simulink model "ASM_Traffic_MultiCore"  (R2026a)
settings: Solver=ode1  StartTime=SIM.tstart.v  StopTime=SIM.tend.v  FixedStep=SIM.StepSize.v
PostLoadFcn:
  | if any(exist('dsrtsu_mdlpostloadfcn', 'file') ~= 0), dsrtsu_mdlpostloadfcn('Execute', bdroot); end
  | try, asm_mdl_postloadfcn(bdroot, 'UpdateModel', 3600); catch, disp(lasterr); end,
InitFcn:
  | , if any(exist('rtifpga_mdlclblib', 'file') ~= 0), rtifpga_mdlclblib('Init', bdroot); end,
  | , if any(exist('dsmpb_private', 'file') ~= 0), dsmpb_private('dsmpb_mdlclblib', 'Init', bdroot); end,
model workspace (MAT data in the model file):
  asmReferencePath = [0 0.01 0.02 0.03 0.04 0.05 0.06 0.07 0.08 0.09 0.1 0.11 ... (350007 elements, 50001x7)]
  roadBounds : Simulink.Parameter (value not decoded)
  safetyAxes : Simulink.Parameter (value not decoded)
undefined symbols (not defined in the file): _to_, a0b2, ASM_BrakeHydraulics_DemoSystems, ASM_VehicleDynamics_DemoSystems, b98103fe8ad365046cd0, BrakeCircuit, controllerConfig, CPT, Crankshaft, DiscIntNeverNeededParam, dsmsi, FinalDriveAssembly, MDL, ModeSignals, mu, Pos_BrakePedal_Maneuver, rad, RefSignals, roadFamilyData, roadFamilyId, s_to_rpm, SIM, SoftECU, Suspension, Tire, Transmission
libraries: ASM_Traffic_lib x135, simulink x98, ASM_Utils_lib x77, ASM_VehicleDynamics_lib x70, ASM_Environment_lib x22, dsmpblib x20, dsmsilib x15, MDLD_Utils_lib x10, ASM_BrakeHydraulics_lib x3, sl_discontinuities x2
(part 58 of 65)

== system ASM_Traffic_MultiCore/Environment/Sensors/PlantModel/Object_Sensor_2D/ObjectData/Sensor6/Object_Custom_Values ==
  TrafficObject_Type[] : Inport
  TrafficObject_Type_Data[] : Inport  Port=2
  CUSTOM_SENSOR_OUTPUT : ASM_Traffic_lib/Sensors/Custom_Sensor/CUSTOM_SENSOR_OUTPUT  Tag=ASM_SUBCOMPONENT  ASMProperties=struct('Name','CUSTOM_SENSOR_OUTPUT','Version','5.0','Library','ASM_Traffic_lib')  ASMInstanceName=custom_sensor_output  ASMInstanceID=26
      settings: AttributesFormatString=Instance Name: %<ASMInstanceName>\nInstance ID: %<ASMInstanceID>
  CUSTOM_SENSOR_OUTPUT1 : ASM_Traffic_lib/Sensors/Custom_Sensor/CUSTOM_SENSOR_OUTPUT  Tag=ASM_SUBCOMPONENT  ASMProperties=struct('Name','CUSTOM_SENSOR_OUTPUT','Version','5.0','Library','ASM_Traffic_lib')  ASMInstanceName=custom_sensor_output  ASMInstanceID=27
      settings: AttributesFormatString=Instance Name: %<ASMInstanceName>\nInstance ID: %<ASMInstanceID>
  CUSTOM_SENSOR_OUTPUT2 : ASM_Traffic_lib/Sensors/Custom_Sensor/CUSTOM_SENSOR_OUTPUT  Tag=ASM_SUBCOMPONENT  ASMProperties=struct('Name','CUSTOM_SENSOR_OUTPUT','Version','5.0','Library','ASM_Traffic_lib')  ASMInstanceName=custom_sensor_output  ASMInstanceID=28
      settings: AttributesFormatString=Instance Name: %<ASMInstanceName>\nInstance ID: %<ASMInstanceID>
  Terminator : Terminator
  Terminator1 : Terminator
  Terminator2 : Terminator
  Vectorize_Signals : Subsystem
  "[11:15]" : Selector  IndexOptions=Index vector (dialog)  Indices=[11:15]  OutputSizes=1
  "[1:5]" : Selector  IndexOptions=Index vector (dialog)  Indices=[1:5]  OutputSizes=1
  "[6:10]" : Selector  IndexOptions=Index vector (dialog)  Indices=[6:10]  OutputSizes=1
  Object_Custom_Values[] : Outport  VectorParamsAs1DForOutWhenUnconnected=off
  wires:
  CUSTOM_SENSOR_OUTPUT2/2 -> Vectorize_Signals/3(SensorOutput3)
  CUSTOM_SENSOR_OUTPUT1/2 -> Vectorize_Signals/2(SensorOutput2)
  Vectorize_Signals/1(Vectorized_Custom_Values) -> Object_Custom_Values[]/1
  CUSTOM_SENSOR_OUTPUT/2 -> Vectorize_Signals/1(SensorOutput1)
  CUSTOM_SENSOR_OUTPUT2/1 -> Terminator2/1
  CUSTOM_SENSOR_OUTPUT1/1 -> Terminator1/1
  CUSTOM_SENSOR_OUTPUT/1 -> Terminator/1
  "[6:10]"/1 -> CUSTOM_SENSOR_OUTPUT1/1
  TrafficObject_Type[]/1 -> "[11:15]"/1, "[6:10]"/1, "[1:5]"/1
  TrafficObject_Type_Data[]/1 -> CUSTOM_SENSOR_OUTPUT2/2, CUSTOM_SENSOR_OUTPUT1/2, CUSTOM_SENSOR_OUTPUT/2
  "[1:5]"/1 -> CUSTOM_SENSOR_OUTPUT/1
  "[11:15]"/1 -> CUSTOM_SENSOR_OUTPUT2/1

== system ASM_Traffic_MultiCore/Environment/Sensors/PlantModel/Object_Sensor_2D/ObjectData/Sensor7/ASMSignalCollector ==
  Object_Positions : Inport
  Object_Properties_Box : Inport  Port=2
  Object_Custom_Values : Inport  Port=3
  Bus Creator1 : BusCreator  Inputs=3
  Bus Selector : BusSelector  OutputSignals=Object_Positions
  Bus Selector1 : BusSelector  OutputSignals=Object_Properties_Box
  ASMSignalBus : Outport  VectorParamsAs1DForOutWhenUnconnected=off
  wires:
  Object_Positions/1 -> Bus Selector/1
  Object_Custom_Values/1 -> Bus Creator1/3
  Bus Creator1/1 -> ASMSignalBus/1  "ObjectData"
  Object_Properties_Box/1 -> Bus Selector1/1
  Bus Selector/1 -> Bus Creator1/1  "<Object_Positions>"
  Bus Selector1/1 -> Bus Creator1/2  "<Object_Properties_Box>"

== system ASM_Traffic_MultiCore/Environment/Sensors/PlantModel/Object_Sensor_2D/ObjectData/Sensor7/GetFellowPositionVector ==
  <FellowPositions> : Inport
  Bus Selector11 : BusSelector  OutputSignals=Pos_Fellows_MainPnt_CoorSys_E[x;y;z][m].Pos_x_Fellows[m],Pos_Fellows_MainPnt_CoorSys_E[x;y;z][m].Pos_y_Fellows[m],Pos_Fellows_MainPnt_CoorSys_E[x;y;z][m].Pos_z_Fellows[m],Angle_Fellows[x;y;z][deg].Angle_Roll_Fellows[deg],Angle_Fellows[x;y;z][deg].Angle_Pitch_Fellows[deg],Angle_Fellows[x;y;z][deg].Angle_Yaw_Fellows[deg]
  Mux1 : Mux  Inputs=3
  Mux2 : Mux  Inputs=3
  Pos_Fellows_MainPnt_CoorSys_E[x;y;z][m] : Outport  VectorParamsAs1DForOutWhenUnconnected=off
  Angle_Fellows[deg] : Outport  Port=2  VectorParamsAs1DForOutWhenUnconnected=off
  wires:
  Mux2/1 -> Pos_Fellows_MainPnt_CoorSys_E[x;y;z][m]/1  "Pos_Fellows_MainPnt_CoorSys_E[x;y;z][m]"
  Mux1/1 -> Angle_Fellows[deg]/1  "Pos_Fellows_MainPnt_CoorSys_E_vec"
  Bus Selector11/4 -> Mux1/1  "<Angle_Roll_Fellows[deg]>"
  Bus Selector11/1 -> Mux2/1  "<Pos_x_Fellows[m]>"
  Bus Selector11/2 -> Mux2/2  "<Pos_y_Fellows[m]>"
  Bus Selector11/6 -> Mux1/3  "<Angle_Yaw_Fellows[deg]>"
  Bus Selector11/5 -> Mux1/2  "<Angle_Pitch_Fellows[deg]>"
  <FellowPositions>/1 -> Bus Selector11/1
  Bus Selector11/3 -> Mux2/3  "<Pos_z_Fellows[m]>"

== system ASM_Traffic_MultiCore/Environment/Sensors/PlantModel/Object_Sensor_2D/ObjectData/Sensor7/Object_Custom_Values ==
  TrafficObject_Type[] : Inport
  TrafficObject_Type_Data[] : Inport  Port=2
  CUSTOM_SENSOR_OUTPUT : ASM_Traffic_lib/Sensors/Custom_Sensor/CUSTOM_SENSOR_OUTPUT  Tag=ASM_SUBCOMPONENT  ASMProperties=struct('Name','CUSTOM_SENSOR_OUTPUT','Version','5.0','Library','ASM_Traffic_lib')  ASMInstanceName=custom_sensor_output  ASMInstanceID=29
      settings: AttributesFormatString=Instance Name: %<ASMInstanceName>\nInstance ID: %<ASMInstanceID>
  CUSTOM_SENSOR_OUTPUT1 : ASM_Traffic_lib/Sensors/Custom_Sensor/CUSTOM_SENSOR_OUTPUT  Tag=ASM_SUBCOMPONENT  ASMProperties=struct('Name','CUSTOM_SENSOR_OUTPUT','Version','5.0','Library','ASM_Traffic_lib')  ASMInstanceName=custom_sensor_output  ASMInstanceID=30
      settings: AttributesFormatString=Instance Name: %<ASMInstanceName>\nInstance ID: %<ASMInstanceID>
  CUSTOM_SENSOR_OUTPUT2 : ASM_Traffic_lib/Sensors/Custom_Sensor/CUSTOM_SENSOR_OUTPUT  Tag=ASM_SUBCOMPONENT  ASMProperties=struct('Name','CUSTOM_SENSOR_OUTPUT','Version','5.0','Library','ASM_Traffic_lib')  ASMInstanceName=custom_sensor_output  ASMInstanceID=31
      settings: AttributesFormatString=Instance Name: %<ASMInstanceName>\nInstance ID: %<ASMInstanceID>
  Terminator : Terminator
  Terminator1 : Terminator
  Terminator2 : Terminator
  Vectorize_Signals : Subsystem
  "[11:15]" : Selector  IndexOptions=Index vector (dialog)  Indices=[11:15]  OutputSizes=1
  "[1:5]" : Selector  IndexOptions=Index vector (dialog)  Indices=[1:5]  OutputSizes=1
  "[6:10]" : Selector  IndexOptions=Index vector (dialog)  Indices=[6:10]  OutputSizes=1
  Object_Custom_Values[] : Outport  VectorParamsAs1DForOutWhenUnconnected=off
  wires:
  "[11:15]"/1 -> CUSTOM_SENSOR_OUTPUT2/1
  "[1:5]"/1 -> CUSTOM_SENSOR_OUTPUT/1
  TrafficObject_Type_Data[]/1 -> CUSTOM_SENSOR_OUTPUT1/2, CUSTOM_SENSOR_OUTPUT2/2, CUSTOM_SENSOR_OUTPUT/2
  TrafficObject_Type[]/1 -> "[11:15]"/1, "[6:10]"/1, "[1:5]"/1
  "[6:10]"/1 -> CUSTOM_SENSOR_OUTPUT1/1
  CUSTOM_SENSOR_OUTPUT/1 -> Terminator/1
  CUSTOM_SENSOR_OUTPUT1/1 -> Terminator1/1
  CUSTOM_SENSOR_OUTPUT2/1 -> Terminator2/1
  CUSTOM_SENSOR_OUTPUT/2 -> Vectorize_Signals/1(SensorOutput1)
  Vectorize_Signals/1(Vectorized_Custom_Values) -> Object_Custom_Values[]/1
  CUSTOM_SENSOR_OUTPUT1/2 -> Vectorize_Signals/2(SensorOutput2)
  CUSTOM_SENSOR_OUTPUT2/2 -> Vectorize_Signals/3(SensorOutput3)

== system ASM_Traffic_MultiCore/Environment/Sensors/PlantModel/Object_Sensor_3D/CustomPoints/Sensor1/CustomPoints ==
  Sensor_Idx[] : Inport
  Sensor_Data[] : Inport  Port=2
  Enable : EnablePort
  Bus Creator2 : BusCreator  Inputs=19
  CUSTOM_POINTS_1 : ASM_Traffic_lib/Sensors/Custom Points/CUSTOM_POINTS  Tag=ASM_SUBCOMPONENT  Sw_Visible_Points_Filter_Enable=MDL.Traffic.Sensors.CustomPoints_1.Sw_Visible_Points_Filter_Enable  Sw_Sort_Enable=MDL.Traffic.Sensors.CustomPoints_1.Sw_Sort_Enable  Sw_Sort_Attribute=MDL.Traffic.Sensors.CustomPoints_1.Sw_Sort_Attribute  Sw_Sort_Direction=MDL.Traffic.Sensors.CustomPoints_1.Sw_Sort_Direction  ASMProperties=struct('Name','CUSTOM_POINTS','Version','2.0','Library','ASM_Traffic_lib')  ASMInstanceName=custom_points  ASMInstanceID=1  Const_Output_Dimension_Objects=MDL.Traffic.Sensors.CustomPoints_1.Const_Output_Dimension_Objects  Const_Output_Dimension_Object_Points=MDL.Traffic.Sensors.CustomPoints_1.Const_Output_Dimension_Object_Points
  MODELDESK_GROUP : ASM_Utils_lib/ModelDeskInterface/MODELDESK_GROUP  MDLDGroup=Object Sensor 3D 1  ASMProperties=struct('Name','MODELDESK_GROUP','Version','1.0','Library','ASM_Utils_lib')
  Terminator : Terminator
  CustomPoint_Signals[] : Outport  OutputWhenDisabled=reset  InitialOutput=[0]  VectorParamsAs1DForOutWhenUnconnected=off
  wires:
  CUSTOM_POINTS_1/20 -> Bus Creator2/19  "Object_Type[]"
  CUSTOM_POINTS_1/19 -> Bus Creator2/18  "Object_ID[]"
  CUSTOM_POINTS_1/18 -> Bus Creator2/17  "Data_5[]"
  CUSTOM_POINTS_1/17 -> Bus Creator2/16  "Data_4[]"
  CUSTOM_POINTS_1/16 -> Bus Creator2/15  "Data_3[]"
  CUSTOM_POINTS_1/15 -> Bus Creator2/14  "Data_2[]"
  CUSTOM_POINTS_1/14 -> Bus Creator2/13  "Data_1[]"
  CUSTOM_POINTS_1/13 -> Bus Creator2/12  "Angle_Ver_CoorSys_S[deg]"
  CUSTOM_POINTS_1/12 -> Bus Creator2/11  "Angle_Hor_CoorSys_S[deg]"
  CUSTOM_POINTS_1/11 -> Bus Creator2/10  "Pos_CoorSys_E[x;y;z][m]"
  CUSTOM_POINTS_1/10 -> Bus Creator2/9  "Pos_CoorSys_S[x;y;z][m]"
  CUSTOM_POINTS_1/9 -> Bus Creator2/8  "a_CoorSys_S[x;y;z][m|s2]"
  CUSTOM_POINTS_1/8 -> Bus Creator2/7  "a_CoorSys_S[m|s2]"
  CUSTOM_POINTS_1/7 -> Bus Creator2/6  "v_CoorSys_S[x;y;z][m|s]"
  CUSTOM_POINTS_1/6 -> Bus Creator2/5  "v_CoorSys_S[m|s]"
  CUSTOM_POINTS_1/5 -> Bus Creator2/4  "Dist_CoorSys_S[m]"
  CUSTOM_POINTS_1/4 -> Bus Creator2/3  "ID[]"
  CUSTOM_POINTS_1/3 -> Bus Creator2/2  "Flag_Is_Occluded[0|1]"
  CUSTOM_POINTS_1/2 -> Bus Creator2/1  "Flag_In_Scope[0|1]"
  Bus Creator2/1 -> CustomPoint_Signals[]/1
  CUSTOM_POINTS_1/1 -> Terminator/1
  Sensor_Idx[]/1 -> CUSTOM_POINTS_1/1
  Sensor_Data[]/1 -> CUSTOM_POINTS_1/2

== system ASM_Traffic_MultiCore/Environment/Sensors/PlantModel/Object_Sensor_3D/CustomPoints/Sensor1/CustomPointsOutput ==
  SensorSchedulingEnable[0|1] : Inport
  SensorActive[0|1] : Inport  Port=2
  SensorEnable[0|1] : Inport  Port=3
  DelayPulse[0|1] : Inport  Port=4
  CustomPoints_Signals_In[] : Inport  Port=5
  CUSTOM_POINTS_SIGNALS_DELAY_1 : ASM_Traffic_lib/Sensors/Custom Points/CUSTOM_POINTS_SIGNALS_DELAY  ASMProperties=struct('Name','CUSTOM_POINTS_SIGNALS_DELAY','Version','2.0','Library','ASM_Traffic_lib')  ASMInstanceName=custom_points_signals_delay  ASMInstanceID=1
  HoldSignals : Subsystem
  Logical Operator1 : Logic  Operator=OR  AllPortsSameDT=off  OutDataTypeStr=boolean
  ResetPulse : Subsystem
  SignalBus : Subsystem
  CustomPoints_Signals_Out[] : Outport  VectorParamsAs1DForOutWhenUnconnected=off
  wires:
  ResetPulse/1(ResetPulse[0|1]) -> Logical Operator1/1, HoldSignals/1(ResetPulse[0|1]), CUSTOM_POINTS_SIGNALS_DELAY_1/1
  SensorEnable[0|1]/1 -> Logical Operator1/2
  Logical Operator1/1 -> HoldSignals/Enable
  SensorActive[0|1]/1 -> ResetPulse/2(SensorActive[0|1])
  HoldSignals/1(CustomPoints_Signals_Out[]) -> CUSTOM_POINTS_SIGNALS_DELAY_1/3
  SignalBus/1(CustomPoints_Signals_Out[]) -> CustomPoints_Signals_Out[]/1
  DelayPulse[0|1]/1 -> CUSTOM_POINTS_SIGNALS_DELAY_1/2
  CUSTOM_POINTS_SIGNALS_DELAY_1/1 -> SignalBus/1(CustomPoints_Signals_In[])
  CustomPoints_Signals_In[]/1 -> HoldSignals/2(CustomPoints_Signals_In[])
  SensorSchedulingEnable[0|1]/1 -> ResetPulse/1(Enable[0|1])

== system ASM_Traffic_MultiCore/Environment/Sensors/PlantModel/Object_Sensor_3D/CustomPoints/Sensor2/CustomPoints ==
  Sensor_Idx[] : Inport
  Sensor_Data[] : Inport  Port=2
  Enable : EnablePort
  Bus Creator2 : BusCreator  Inputs=19
  CUSTOM_POINTS_2 : ASM_Traffic_lib/Sensors/Custom Points/CUSTOM_POINTS  Tag=ASM_SUBCOMPONENT  Sw_Visible_Points_Filter_Enable=MDL.Traffic.Sensors.CustomPoints_2.Sw_Visible_Points_Filter_Enable  Sw_Sort_Enable=MDL.Traffic.Sensors.CustomPoints_2.Sw_Sort_Enable  Sw_Sort_Attribute=MDL.Traffic.Sensors.CustomPoints_2.Sw_Sort_Attribute  Sw_Sort_Direction=MDL.Traffic.Sensors.CustomPoints_2.Sw_Sort_Direction  ASMProperties=struct('Name','CUSTOM_POINTS','Version','2.0','Library','ASM_Traffic_lib')  ASMInstanceName=custom_points  ASMInstanceID=2  Const_Output_Dimension_Objects=MDL.Traffic.Sensors.CustomPoints_2.Const_Output_Dimension_Objects  Const_Output_Dimension_Object_Points=MDL.Traffic.Sensors.CustomPoints_2.Const_Output_Dimension_Object_Points
      settings: AttributesFormatString=Instance Name: %<ASMInstanceName>\nInstance ID: %<ASMInstanceID>
  MODELDESK_GROUP : ASM_Utils_lib/ModelDeskInterface/MODELDESK_GROUP  MDLDGroup=Object Sensor 3D 2  ASMProperties=struct('Name','MODELDESK_GROUP','Version','1.0','Library','ASM_Utils_lib')
  Terminator : Terminator
  CustomPoint_Signals[] : Outport  OutputWhenDisabled=reset  InitialOutput=[0]  VectorParamsAs1DForOutWhenUnconnected=off
  wires:
  CUSTOM_POINTS_2/3 -> Bus Creator2/2  "Flag_Is_Occluded[0|1]"
  CUSTOM_POINTS_2/11 -> Bus Creator2/10  "Pos_CoorSys_E[x;y;z][m]"
  CUSTOM_POINTS_2/8 -> Bus Creator2/7  "a_CoorSys_S[m|s2]"
  CUSTOM_POINTS_2/5 -> Bus Creator2/4  "Dist_CoorSys_S[m]"
  CUSTOM_POINTS_2/4 -> Bus Creator2/3  "ID[]"
  CUSTOM_POINTS_2/13 -> Bus Creator2/12  "Angle_Ver_CoorSys_S[deg]"
  CUSTOM_POINTS_2/6 -> Bus Creator2/5  "v_CoorSys_S[m|s]"
  CUSTOM_POINTS_2/7 -> Bus Creator2/6  "v_CoorSys_S[x;y;z][m|s]"
  CUSTOM_POINTS_2/15 -> Bus Creator2/14  "Data_2[]"
  CUSTOM_POINTS_2/16 -> Bus Creator2/15  "Data_3[]"
  CUSTOM_POINTS_2/14 -> Bus Creator2/13  "Data_1[]"
  CUSTOM_POINTS_2/10 -> Bus Creator2/9  "Pos_CoorSys_S[x;y;z][m]"
  CUSTOM_POINTS_2/12 -> Bus Creator2/11  "Angle_Hor_CoorSys_S[deg]"
  CUSTOM_POINTS_2/18 -> Bus Creator2/17  "Data_5[]"
  CUSTOM_POINTS_2/17 -> Bus Creator2/16  "Data_4[]"
  Bus Creator2/1 -> CustomPoint_Signals[]/1
  CUSTOM_POINTS_2/2 -> Bus Creator2/1  "Flag_In_Scope[0|1]"
  CUSTOM_POINTS_2/9 -> Bus Creator2/8  "a_CoorSys_S[x;y;z][m|s2]"
  CUSTOM_POINTS_2/19 -> Bus Creator2/18  "Object_ID[]"
  CUSTOM_POINTS_2/20 -> Bus Creator2/19  "Object_Type[]"
  Sensor_Data[]/1 -> CUSTOM_POINTS_2/2
  Sensor_Idx[]/1 -> CUSTOM_POINTS_2/1
  CUSTOM_POINTS_2/1 -> Terminator/1

== system ASM_Traffic_MultiCore/Environment/Sensors/PlantModel/Object_Sensor_3D/CustomPoints/Sensor2/CustomPointsOutput ==
  SensorSchedulingEnable[0|1] : Inport
  SensorActive[0|1] : Inport  Port=2
  SensorEnable[0|1] : Inport  Port=3
  DelayPulse[0|1] : Inport  Port=4
  CustomPoint_Signals_In[] : Inport  Port=5
  CUSTOM_POINTS_SIGNALS_DELAY_2 : ASM_Traffic_lib/Sensors/Custom Points/CUSTOM_POINTS_SIGNALS_DELAY  ASMProperties=struct('Name','CUSTOM_POINTS_SIGNALS_DELAY','Version','2.0','Library','ASM_Traffic_lib')  ASMInstanceName=custom_points_signals_delay  ASMInstanceID=1
  HoldSignals : Subsystem
  Logical Operator1 : Logic  Operator=OR  AllPortsSameDT=off  OutDataTypeStr=boolean
  ResetPulse : Subsystem
  SignalBus : Subsystem
  CustomPoints_Signals_Out[] : Outport  VectorParamsAs1DForOutWhenUnconnected=off
  wires:
  SensorActive[0|1]/1 -> ResetPulse/2(SensorActive[0|1])
  ResetPulse/1(ResetPulse[0|1]) -> Logical Operator1/1, HoldSignals/1(ResetPulse[0|1]), CUSTOM_POINTS_SIGNALS_DELAY_2/1
  SensorEnable[0|1]/1 -> Logical Operator1/2
  SensorSchedulingEnable[0|1]/1 -> ResetPulse/1(Enable[0|1])
  DelayPulse[0|1]/1 -> CUSTOM_POINTS_SIGNALS_DELAY_2/2
  Logical Operator1/1 -> HoldSignals/Enable
  HoldSignals/1(CustomPoints_Signals_Out[]) -> CUSTOM_POINTS_SIGNALS_DELAY_2/3
  SignalBus/1(CustomPoints_Signals_Out[]) -> CustomPoints_Signals_Out[]/1
  CUSTOM_POINTS_SIGNALS_DELAY_2/1 -> SignalBus/1(CustomPoints_Signals_In[])
  CustomPoint_Signals_In[]/1 -> HoldSignals/2(CustomPoints_Signals_In[])

== system ASM_Traffic_MultiCore/Environment/Sensors/PlantModel/Object_Sensor_3D/CustomPoints/Sensor3/CustomPoints ==
  Sensor_Idx[] : Inport
  Sensor_Data[] : Inport  Port=2
  Enable : EnablePort
  Bus Creator2 : BusCreator  Inputs=19
  CUSTOM_POINTS_3 : ASM_Traffic_lib/Sensors/Custom Points/CUSTOM_POINTS  Tag=ASM_SUBCOMPONENT  Sw_Visible_Points_Filter_Enable=MDL.Traffic.Sensors.CustomPoints_3.Sw_Visible_Points_Filter_Enable  Sw_Sort_Enable=MDL.Traffic.Sensors.CustomPoints_3.Sw_Sort_Enable  Sw_Sort_Attribute=MDL.Traffic.Sensors.CustomPoints_3.Sw_Sort_Attribute  Sw_Sort_Direction=MDL.Traffic.Sensors.CustomPoints_3.Sw_Sort_Direction  ASMProperties=struct('Name','CUSTOM_POINTS','Version','2.0','Library','ASM_Traffic_lib')  ASMInstanceName=custom_points  ASMInstanceID=3  Const_Output_Dimension_Objects=MDL.Traffic.Sensors.CustomPoints_3.Const_Output_Dimension_Objects  Const_Output_Dimension_Object_Points=MDL.Traffic.Sensors.CustomPoints_3.Const_Output_Dimension_Object_Points
      settings: AttributesFormatString=Instance Name: %<ASMInstanceName>\nInstance ID: %<ASMInstanceID>
  MODELDESK_GROUP : ASM_Utils_lib/ModelDeskInterface/MODELDESK_GROUP  MDLDGroup=Object Sensor 3D 3  ASMProperties=struct('Name','MODELDESK_GROUP','Version','1.0','Library','ASM_Utils_lib')
  Terminator : Terminator
  CustomPoint_Signals[] : Outport  OutputWhenDisabled=reset  InitialOutput=[0]  VectorParamsAs1DForOutWhenUnconnected=off
  wires:
  CUSTOM_POINTS_3/3 -> Bus Creator2/2  "Flag_Is_Occluded[0|1]"
  CUSTOM_POINTS_3/11 -> Bus Creator2/10  "Pos_CoorSys_E[x;y;z][m]"
  CUSTOM_POINTS_3/8 -> Bus Creator2/7  "a_CoorSys_S[m|s2]"
  CUSTOM_POINTS_3/5 -> Bus Creator2/4  "Dist_CoorSys_S[m]"
  CUSTOM_POINTS_3/4 -> Bus Creator2/3  "ID[]"
  CUSTOM_POINTS_3/13 -> Bus Creator2/12  "Angle_Ver_CoorSys_S[deg]"
  CUSTOM_POINTS_3/6 -> Bus Creator2/5  "v_CoorSys_S[m|s]"
  CUSTOM_POINTS_3/7 -> Bus Creator2/6  "v_CoorSys_S[x;y;z][m|s]"
  CUSTOM_POINTS_3/15 -> Bus Creator2/14  "Data_2[]"
  CUSTOM_POINTS_3/16 -> Bus Creator2/15  "Data_3[]"
  CUSTOM_POINTS_3/14 -> Bus Creator2/13  "Data_1[]"
  CUSTOM_POINTS_3/10 -> Bus Creator2/9  "Pos_CoorSys_S[x;y;z][m]"
  CUSTOM_POINTS_3/12 -> Bus Creator2/11  "Angle_Hor_CoorSys_S[deg]"
  CUSTOM_POINTS_3/18 -> Bus Creator2/17  "Data_5[]"
  CUSTOM_POINTS_3/17 -> Bus Creator2/16  "Data_4[]"
  Bus Creator2/1 -> CustomPoint_Signals[]/1
  CUSTOM_POINTS_3/2 -> Bus Creator2/1  "Flag_In_Scope[0|1]"
  CUSTOM_POINTS_3/9 -> Bus Creator2/8  "a_CoorSys_S[x;y;z][m|s2]"
  CUSTOM_POINTS_3/19 -> Bus Creator2/18  "Object_ID[]"
  CUSTOM_POINTS_3/20 -> Bus Creator2/19  "Object_Type[]"
  Sensor_Idx[]/1 -> CUSTOM_POINTS_3/1
  Sensor_Data[]/1 -> CUSTOM_POINTS_3/2
  CUSTOM_POINTS_3/1 -> Terminator/1

== system ASM_Traffic_MultiCore/Environment/Sensors/PlantModel/Object_Sensor_3D/CustomPoints/Sensor3/CustomPointsOutput ==
  SensorSchedulingEnable[0|1] : Inport
  SensorActive[0|1] : Inport  Port=2
  SensorEnable[0|1] : Inport  Port=3
  DelayPulse[0|1] : Inport  Port=4
  CustomPoints_Signals_In[] : Inport  Port=5
  CUSTOM_POINTS_SIGNALS_DELAY_3 : ASM_Traffic_lib/Sensors/Custom Points/CUSTOM_POINTS_SIGNALS_DELAY  ASMProperties=struct('Name','CUSTOM_POINTS_SIGNALS_DELAY','Version','2.0','Library','ASM_Traffic_lib')  ASMInstanceName=custom_points_signals_delay  ASMInstanceID=1
  HoldSignals : Subsystem
  Logical Operator1 : Logic  Operator=OR  AllPortsSameDT=off  OutDataTypeStr=boolean
  ResetPulse1 : Subsystem
  SignalBus : Subsystem
  CustomPoints_Signals_Out[] : Outport  VectorParamsAs1DForOutWhenUnconnected=off
  wires:
  DelayPulse[0|1]/1 -> CUSTOM_POINTS_SIGNALS_DELAY_3/2
  SensorActive[0|1]/1 -> ResetPulse1/2(SensorActive[0|1])
  ResetPulse1/1(ResetPulse[0|1]) -> Logical Operator1/1, HoldSignals/1(ResetPulse[0|1]), CUSTOM_POINTS_SIGNALS_DELAY_3/1
  SensorSchedulingEnable[0|1]/1 -> ResetPulse1/1(Enable[0|1])
  SensorEnable[0|1]/1 -> Logical Operator1/2
  HoldSignals/1(CustomPoints_Signals_Out[]) -> CUSTOM_POINTS_SIGNALS_DELAY_3/3
  Logical Operator1/1 -> HoldSignals/Enable
  SignalBus/1(CustomPoints_Signals_Out[]) -> CustomPoints_Signals_Out[]/1
  CUSTOM_POINTS_SIGNALS_DELAY_3/1 -> SignalBus/1(CustomPoints_Signals_In[])
  CustomPoints_Signals_In[]/1 -> HoldSignals/2(CustomPoints_Signals_In[])

== system ASM_Traffic_MultiCore/Environment/Sensors/PlantModel/Object_Sensor_3D/ObjectData/BoundingBoxData_CoorSys_E/BoundingBoxData_CoorSys_E ==
  Object_ID[] : Inport
  Object_Type[] : Inport  Port=2
  Traffic_Signals : Inport  Port=3
  Road_Signals : Inport  Port=4
  Bus Creator1 : BusCreator  Inputs=9
  Bus Selector1 : BusSelector  OutputSignals=Object_Properties_Box.Length_Object[m],Object_Properties_Box.Width_Object[m],Object_Properties_Box.Height_Object[m],Object_Properties_Box.Flag_BoxProperties[0|1]
  Bus Selector2 : BusSelector  OutputSignals=Object_Positions.Angle_x_Objects_CoorSysE[deg],Object_Positions.Angle_y_Objects_CoorSysE[deg],Object_Positions.Angle_z_Objects_CoorSysE[deg]
  Bus Selector3 : BusSelector  OutputSignals=Object_Properties_Box.PosVec_x_CenterPnt_Object[m],Object_Properties_Box.PosVec_y_CenterPnt_Object[m],Object_Properties_Box.PosVec_z_CenterPnt_Object[m]
  Bus Selector4 : BusSelector  OutputSignals=Plant.Road_TrafficFellows.Network_Item_Type_Fellows[],Plant.Road_TrafficFellows.Network_Item_Id_Fellows[],Plant.TrafficObject_Data[]
  Bus Selector5 : BusSelector  OutputSignals=Plant.Traffic_Signals_toEnvironment
  Bus Selector6 : BusSelector  OutputSignals=Plant.ObjectParameters.TrafficObjects.TrafficObject_Type_Data[]
  Bus Selector7 : BusSelector  OutputSignals=Object_Positions.Pos_x_MainPnt_Objects_CoorSysE[m],Object_Positions.Pos_y_MainPnt_Objects_CoorSysE[m],Object_Positions.Pos_z_MainPnt_Objects_CoorSysE[m]
  Bus Selector8 : BusSelector  OutputSignals=Object_Positions.Angle_x_Objects_CoorSysE[deg],Object_Positions.Angle_y_Objects_CoorSysE[deg],Object_Positions.Angle_z_Objects_CoorSysE[deg]
  COORDINATE_TRANSFORMATION_B_TO_A : ASM_Utils_lib/MatrixOperations/COORDINATE_TRANSFORMATION_B_TO_A  ASMLibrary2Check=ASM_Traffic_lib
  GetFellowPositionVector : Subsystem
  OBJECT_POSITION : ASM_Traffic_lib/Objects/OBJECT_POSITION  MaxNumFellows=MDL.Traffic.MaxNumFellows  ASMProperties=struct('Name','OBJECT_POSITION','Version','2.0','Library','ASM_Traffic_lib')  ASMInstanceName=object_position  ASMInstanceID=1
  OBJECT_PROPERTIES_BOX : ASM_Traffic_lib/Objects/OBJECT_PROPERTIES_BOX  ASMProperties=struct('Name','OBJECT_PROPERTIES_BOX','Version','2.0','Library','ASM_Traffic_lib')  ASMInstanceName=object_properties_box  ASMInstanceID=1
  Product{,1..8} (9 alike) : Product
  Terminator : Terminator
  Terminator1 : Terminator
  Boundingboxes : Outport  VectorParamsAs1DForOutWhenUnconnected=off
  wires:
  Bus Selector5/1 -> GetFellowPositionVector/1(<FellowPositions>)  "<Traffic_Signals_toEnvironment>"
  Traffic_Signals/1 -> Bus Selector6/1, Bus Selector5/1
  GetFellowPositionVector/1(Pos_Fellows_MainPnt_CoorSys_E[x;y;z][m]) -> OBJECT_POSITION/2
  GetFellowPositionVector/2(Angle_Fellows[deg]) -> OBJECT_POSITION/3
  Bus Selector1/1 -> Product6/1  "<Length_Object[m]>"
  Bus Selector1/2 -> Product7/1  "<Width_Object[m]>"
  Bus Selector1/3 -> Product8/1  "<Height_Object[m]>"
  Bus Selector1/4 -> Product7/2, Product3/2, Product2/2, Product1/2, Product/2, Product4/2, Product5/2, Product6/2, Product8/2  "<Flag_BoxProperties[0|1]>"
  Product8/1 -> Bus Creator1/9  "Height_Object[m]"
  Product7/1 -> Bus Creator1/8  "Width_Object[m]"
  Product6/1 -> Bus Creator1/7  "Length_Object[m]"
  Product5/1 -> Bus Creator1/6  "Angle_z_Objects_CoorSysE[deg]"
  Product4/1 -> Bus Creator1/5  "Angle_y_Objects_CoorSysE[deg]"
  Product3/1 -> Bus Creator1/4  "Angle_x_Objects_CoorSysE[deg]"
  Product2/1 -> Bus Creator1/3  "Pos_z_CoorSysE[m]"
  Product1/1 -> Bus Creator1/2  "Pos_y_CoorSysE[m]"
  Product/1 -> Bus Creator1/1  "Pos_x_CoorSysE[m]"
  Bus Selector8/1 -> COORDINATE_TRANSFORMATION_B_TO_A/7  "<Angle_x_Objects_CoorSysE[deg]>"
  Bus Selector8/2 -> COORDINATE_TRANSFORMATION_B_TO_A/8  "<Angle_y_Objects_CoorSysE[deg]>"
  Bus Selector8/3 -> COORDINATE_TRANSFORMATION_B_TO_A/9  "<Angle_z_Objects_CoorSysE[deg]>"
  COORDINATE_TRANSFORMATION_B_TO_A/3 -> Product2/1  "Pos_z_CoorSysE[m]"
  COORDINATE_TRANSFORMATION_B_TO_A/2 -> Product1/1  "Pos_y_CoorSysE[m]"
  COORDINATE_TRANSFORMATION_B_TO_A/1 -> Product/1  "Pos_x_CoorSysE[m]"
  Bus Selector2/3 -> Product5/1  "<Angle_z_Objects_CoorSysE[deg]>"
  Bus Selector2/2 -> Product4/1  "<Angle_y_Objects_CoorSysE[deg]>"
  Bus Selector2/1 -> Product3/1  "<Angle_x_Objects_CoorSysE[deg]>"
  Bus Selector7/3 -> COORDINATE_TRANSFORMATION_B_TO_A/3  "<Pos_z_MainPnt_Objects_CoorSysE[m]>"
  Bus Selector7/2 -> COORDINATE_TRANSFORMATION_B_TO_A/2  "<Pos_y_MainPnt_Objects_CoorSysE[m]>"
  Bus Selector7/1 -> COORDINATE_TRANSFORMATION_B_TO_A/1  "<Pos_x_MainPnt_Objects_CoorSysE[m]>"
  Bus Selector3/1 -> COORDINATE_TRANSFORMATION_B_TO_A/4  "<PosVec_x_CenterPnt_Object[m]>"
  Bus Selector3/2 -> COORDINATE_TRANSFORMATION_B_TO_A/5  "<PosVec_y_CenterPnt_Object[m]>"
  Bus Selector3/3 -> COORDINATE_TRANSFORMATION_B_TO_A/6  "<PosVec_z_CenterPnt_Object[m]>"
  Bus Creator1/1 -> Boundingboxes/1  "Boundingboxes_DetectedObjects"
  Object_Type[]/1 -> OBJECT_PROPERTIES_BOX/1
  Object_ID[]/1 -> OBJECT_POSITION/1
  OBJECT_PROPERTIES_BOX/2 -> Bus Selector1/1, Bus Selector3/1
  OBJECT_POSITION/2 -> Bus Selector8/1, Bus Selector2/1, Bus Selector7/1
  Bus Selector6/1 -> OBJECT_PROPERTIES_BOX/2  "<TrafficObject_Type_Data[]>"
  Bus Selector4/3 -> OBJECT_POSITION/6  "<TrafficObject_Data[]>"
  Bus Selector4/2 -> OBJECT_POSITION/5  "<Network_Item_Id_Fellows[]>"
  Bus Selector4/1 -> OBJECT_POSITION/4  "<Network_Item_Type_Fellows[]>"
  Road_Signals/1 -> Bus Selector4/1
  OBJECT_PROPERTIES_BOX/1 -> Terminator1/1
  OBJECT_POSITION/1 -> Terminator/1

== system ASM_Traffic_MultiCore/Environment/Sensors/PlantModel/Object_Sensor_3D/ObjectData/BoundingBoxData_CoorSys_E/Unique_Signals_Sorted ==
  Sensor1_Signals[] : Inport
  Sensor2_Signals[] : Inport  Port=2
  Sensor3_Signals[] : Inport  Port=3
  Bus Selector : BusSelector  OutputSignals=SensorOutput.Dist_Object[m]
  Bus Selector1 : BusSelector  OutputSignals=SensorOutput.Object_ID[]
  Bus Selector10 : BusSelector  OutputSignals=Info.Flag_Object_In_Scope[0Out|1In]
  Bus Selector11 : BusSelector  OutputSignals=Info.Flag_Object_In_Scope[0Out|1In]
  Bus Selector2 : BusSelector  OutputSignals=SensorOutput.Dist_Object[m]
  Bus Selector3 : BusSelector  OutputSignals=SensorOutput.Dist_Object[m]
  Bus Selector4 : BusSelector  OutputSignals=SensorOutput.Object_Type[]
  Bus Selector5 : BusSelector  OutputSignals=SensorOutput.Object_ID[]
  Bus Selector6 : BusSelector  OutputSignals=SensorOutput.Object_ID[]
  Bus Selector7 : BusSelector  OutputSignals=SensorOutput.Object_Type[]
  Bus Selector8 : BusSelector  OutputSignals=SensorOutput.Object_Type[]
  Bus Selector9 : BusSelector  OutputSignals=Info.Flag_Object_In_Scope[0Out|1In]
  DETECTED_OBJECTS_MERGE : ASM_Traffic_lib/Sensors/Utilities/DETECTED_OBJECTS_MERGE  Const_Output_Dimension=MDL.Traffic.Sensors.DetectedObjectsMerge.Const_Output_Dimension  ASMProperties=struct('Name','DETECTED_OBJECTS_MERGE','Version','1.0','Library','ASM_Traffic_lib')  ASMInstanceName=detected_objects_merge  ASMInstanceID=1
  Mux{,1..3} (4 alike) : Mux  Inputs=3
  Terminator : Terminator
  Object_ID[] : Outport  VectorParamsAs1DForOutWhenUnconnected=off
  Object_Type[] : Outport  Port=2  VectorParamsAs1DForOutWhenUnconnected=off
  wires:
  Mux3/1 -> DETECTED_OBJECTS_MERGE/1  "Flag_Object_In_Scope[0Out|1In]"
  Bus Selector10/1 -> Mux3/2  "<Flag_Object_In_Scope[0Out|1In]>"
  Bus Selector11/1 -> Mux3/3  "<Flag_Object_In_Scope[0Out|1In]>"
  Bus Selector9/1 -> Mux3/1  "<Flag_Object_In_Scope[0Out|1In]>"
  DETECTED_OBJECTS_MERGE/3 -> Object_Type[]/1
  DETECTED_OBJECTS_MERGE/2 -> Object_ID[]/1
  DETECTED_OBJECTS_MERGE/1 -> Terminator/1
  Bus Selector1/1 -> Mux1/1  "<Object_ID[]>"
  Bus Selector2/1 -> Mux/2  "<Dist_Object[m]>"
  Bus Selector3/1 -> Mux/3  "<Dist_Object[m]>"
  Bus Selector5/1 -> Mux1/2  "<Object_ID[]>"
  Bus Selector6/1 -> Mux1/3  "<Object_ID[]>"
  Bus Selector4/1 -> Mux2/1  "<Object_Type[]>"
  Bus Selector7/1 -> Mux2/2  "<Object_Type[]>"
  Bus Selector8/1 -> Mux2/3  "<Object_Type[]>"
  Sensor2_Signals[]/1 -> Bus Selector2/1, Bus Selector5/1, Bus Selector7/1, Bus Selector10/1
  Mux1/1 -> DETECTED_OBJECTS_MERGE/3  "Object_ID[]"
  Sensor1_Signals[]/1 -> Bus Selector9/1, Bus Selector/1, Bus Selector1/1, Bus Selector4/1
  Sensor3_Signals[]/1 -> Bus Selector3/1, Bus Selector8/1, Bus Selector6/1, Bus Selector11/1
  Bus Selector/1 -> Mux/1  "<Dist_Object[m]>"
  Mux2/1 -> DETECTED_OBJECTS_MERGE/4  "Object_Type[]"
  Mux/1 -> DETECTED_OBJECTS_MERGE/2  "Dist_Object[m]"

== system ASM_Traffic_MultiCore/Environment/Sensors/PlantModel/Object_Sensor_3D/ObjectData/BoundingBoxData_CoorSys_E/avoid_incomplete_trace2source ==
  In1 : Inport
  DummyGain : Gain
  Out1 : Outport
  wires:
  In1/1 -> DummyGain/1
  DummyGain/1 -> Out1/1

== system ASM_Traffic_MultiCore/Environment/Sensors/PlantModel/Object_Sensor_3D/ObjectData/BoundingBoxData_CoorSys_E/avoid_incomplete_trace2source1 ==
  In1 : Inport
  DummyGain : Gain
  Out1 : Outport
  wires:
  DummyGain/1 -> Out1/1
  In1/1 -> DummyGain/1

== system ASM_Traffic_MultiCore/Environment/Sensors/PlantModel/Object_Sensor_3D/ObjectData/Sensor1/ASMSignalCollector ==
  Object_Positions : Inport
  Object_Properties_Box : Inport  Port=2
  Object_Custom_Values : Inport  Port=3
  Bus Creator1 : BusCreator  Inputs=3
  Bus Selector : BusSelector  OutputSignals=Object_Positions
  Bus Selector1 : BusSelector  OutputSignals=Object_Properties_Box
  ASMSignalBus : Outport  VectorParamsAs1DForOutWhenUnconnected=off
  wires:
  Object_Positions/1 -> Bus Selector/1
  Object_Custom_Values/1 -> Bus Creator1/3
  Bus Creator1/1 -> ASMSignalBus/1  "ObjectData"
  Object_Properties_Box/1 -> Bus Selector1/1
  Bus Selector/1 -> Bus Creator1/1  "<Object_Positions>"
  Bus Selector1/1 -> Bus Creator1/2  "<Object_Properties_Box>"

== system ASM_Traffic_MultiCore/Environment/Sensors/PlantModel/Object_Sensor_3D/ObjectData/Sensor1/GetFellowPositionVector ==
  <FellowPositions> : Inport
  Bus Selector11 : BusSelector  OutputSignals=Pos_Fellows_MainPnt_CoorSys_E[x;y;z][m].Pos_x_Fellows[m],Pos_Fellows_MainPnt_CoorSys_E[x;y;z][m].Pos_y_Fellows[m],Pos_Fellows_MainPnt_CoorSys_E[x;y;z][m].Pos_z_Fellows[m],Angle_Fellows[x;y;z][deg].Angle_Roll_Fellows[deg],Angle_Fellows[x;y;z][deg].Angle_Pitch_Fellows[deg],Angle_Fellows[x;y;z][deg].Angle_Yaw_Fellows[deg]
  Mux1 : Mux  Inputs=3
  Mux2 : Mux  Inputs=3
  Pos_Fellows_MainPnt_CoorSys_E[x;y;z][m] : Outport  VectorParamsAs1DForOutWhenUnconnected=off
  Angle_Fellows[deg] : Outport  Port=2  VectorParamsAs1DForOutWhenUnconnected=off
  wires:
  Mux2/1 -> Pos_Fellows_MainPnt_CoorSys_E[x;y;z][m]/1  "Pos_Fellows_MainPnt_CoorSys_E[x;y;z][m]"
  Mux1/1 -> Angle_Fellows[deg]/1  "Pos_Fellows_MainPnt_CoorSys_E_vec"
  Bus Selector11/4 -> Mux1/1  "<Angle_Roll_Fellows[deg]>"
  Bus Selector11/1 -> Mux2/1  "<Pos_x_Fellows[m]>"
  Bus Selector11/2 -> Mux2/2  "<Pos_y_Fellows[m]>"
  Bus Selector11/6 -> Mux1/3  "<Angle_Yaw_Fellows[deg]>"
  Bus Selector11/5 -> Mux1/2  "<Angle_Pitch_Fellows[deg]>"
  <FellowPositions>/1 -> Bus Selector11/1
  Bus Selector11/3 -> Mux2/3  "<Pos_z_Fellows[m]>"

== system ASM_Traffic_MultiCore/Environment/Sensors/PlantModel/Object_Sensor_3D/ObjectData/Sensor1/Object_Custom_Values ==
  TrafficObject_Type[] : Inport
  TrafficObject_Type_Data[] : Inport  Port=2
  CUSTOM_SENSOR_OUTPUT : ASM_Traffic_lib/Sensors/Custom_Sensor/CUSTOM_SENSOR_OUTPUT  Tag=ASM_SUBCOMPONENT  ASMProperties=struct('Name','CUSTOM_SENSOR_OUTPUT','Version','5.0','Library','ASM_Traffic_lib')  ASMInstanceName=custom_sensor_output  ASMInstanceID=2
      settings: AttributesFormatString=Instance Name: %<ASMInstanceName>\nInstance ID: %<ASMInstanceID>
  CUSTOM_SENSOR_OUTPUT1 : ASM_Traffic_lib/Sensors/Custom_Sensor/CUSTOM_SENSOR_OUTPUT  Tag=ASM_SUBCOMPONENT  ASMProperties=struct('Name','CUSTOM_SENSOR_OUTPUT','Version','5.0','Library','ASM_Traffic_lib')  ASMInstanceName=custom_sensor_output  ASMInstanceID=3
      settings: AttributesFormatString=Instance Name: %<ASMInstanceName>\nInstance ID: %<ASMInstanceID>
  CUSTOM_SENSOR_OUTPUT2 : ASM_Traffic_lib/Sensors/Custom_Sensor/CUSTOM_SENSOR_OUTPUT  Tag=ASM_SUBCOMPONENT  ASMProperties=struct('Name','CUSTOM_SENSOR_OUTPUT','Version','5.0','Library','ASM_Traffic_lib')  ASMInstanceName=custom_sensor_output  ASMInstanceID=4
      settings: AttributesFormatString=Instance Name: %<ASMInstanceName>\nInstance ID: %<ASMInstanceID>
  Terminator : Terminator
  Terminator1 : Terminator
  Terminator2 : Terminator
  Vectorize_Signals : Subsystem
  "[11:15]" : Selector  IndexOptions=Index vector (dialog)  Indices=[11:15]  OutputSizes=1
  "[1:5]" : Selector  IndexOptions=Index vector (dialog)  Indices=[1:5]  OutputSizes=1
  "[6:10]" : Selector  IndexOptions=Index vector (dialog)  Indices=[6:10]  OutputSizes=1
  Object_Custom_Values[] : Outport  VectorParamsAs1DForOutWhenUnconnected=off
  wires:
  CUSTOM_SENSOR_OUTPUT2/1 -> Terminator2/1
  CUSTOM_SENSOR_OUTPUT1/1 -> Terminator1/1
  CUSTOM_SENSOR_OUTPUT/1 -> Terminator/1
  Vectorize_Signals/1(Vectorized_Custom_Values) -> Object_Custom_Values[]/1
  CUSTOM_SENSOR_OUTPUT2/2 -> Vectorize_Signals/3(SensorOutput3)
  CUSTOM_SENSOR_OUTPUT1/2 -> Vectorize_Signals/2(SensorOutput2)
  CUSTOM_SENSOR_OUTPUT/2 -> Vectorize_Signals/1(SensorOutput1)
  "[6:10]"/1 -> CUSTOM_SENSOR_OUTPUT1/1
  TrafficObject_Type[]/1 -> "[1:5]"/1, "[6:10]"/1, "[11:15]"/1
  TrafficObject_Type_Data[]/1 -> CUSTOM_SENSOR_OUTPUT2/2, CUSTOM_SENSOR_OUTPUT1/2, CUSTOM_SENSOR_OUTPUT/2
  "[1:5]"/1 -> CUSTOM_SENSOR_OUTPUT/1
  "[11:15]"/1 -> CUSTOM_SENSOR_OUTPUT2/1

== system ASM_Traffic_MultiCore/Environment/Sensors/PlantModel/Object_Sensor_3D/ObjectData/Sensor2/ASMSignalCollector ==
  Object_Positions : Inport
  Object_Properties_Box : Inport  Port=2
  Object_Custom_Values : Inport  Port=3
  Bus Creator1 : BusCreator  Inputs=3
  Bus Selector : BusSelector  OutputSignals=Object_Positions
  Bus Selector1 : BusSelector  OutputSignals=Object_Properties_Box
  ASMSignalBus : Outport  VectorParamsAs1DForOutWhenUnconnected=off
  wires:
  Object_Positions/1 -> Bus Selector/1
  Object_Custom_Values/1 -> Bus Creator1/3
  Bus Creator1/1 -> ASMSignalBus/1  "ObjectData"
  Object_Properties_Box/1 -> Bus Selector1/1
  Bus Selector/1 -> Bus Creator1/1  "<Object_Positions>"
  Bus Selector1/1 -> Bus Creator1/2  "<Object_Properties_Box>"

== system ASM_Traffic_MultiCore/Environment/Sensors/PlantModel/Object_Sensor_3D/ObjectData/Sensor2/GetFellowPositionVector ==
  <FellowPositions> : Inport
  Bus Selector11 : BusSelector  OutputSignals=Pos_Fellows_MainPnt_CoorSys_E[x;y;z][m].Pos_x_Fellows[m],Pos_Fellows_MainPnt_CoorSys_E[x;y;z][m].Pos_y_Fellows[m],Pos_Fellows_MainPnt_CoorSys_E[x;y;z][m].Pos_z_Fellows[m],Angle_Fellows[x;y;z][deg].Angle_Roll_Fellows[deg],Angle_Fellows[x;y;z][deg].Angle_Pitch_Fellows[deg],Angle_Fellows[x;y;z][deg].Angle_Yaw_Fellows[deg]
  Mux1 : Mux  Inputs=3
  Mux2 : Mux  Inputs=3
  Pos_Fellows_MainPnt_CoorSys_E[x;y;z][m] : Outport  VectorParamsAs1DForOutWhenUnconnected=off
  Angle_Fellows[deg] : Outport  Port=2  VectorParamsAs1DForOutWhenUnconnected=off
  wires:
  Mux2/1 -> Pos_Fellows_MainPnt_CoorSys_E[x;y;z][m]/1  "Pos_Fellows_MainPnt_CoorSys_E[x;y;z][m]"
  Mux1/1 -> Angle_Fellows[deg]/1  "Pos_Fellows_MainPnt_CoorSys_E_vec"
  Bus Selector11/4 -> Mux1/1  "<Angle_Roll_Fellows[deg]>"
  Bus Selector11/1 -> Mux2/1  "<Pos_x_Fellows[m]>"
  Bus Selector11/2 -> Mux2/2  "<Pos_y_Fellows[m]>"
  Bus Selector11/6 -> Mux1/3  "<Angle_Yaw_Fellows[deg]>"
  Bus Selector11/5 -> Mux1/2  "<Angle_Pitch_Fellows[deg]>"
  <FellowPositions>/1 -> Bus Selector11/1
  Bus Selector11/3 -> Mux2/3  "<Pos_z_Fellows[m]>"

== system ASM_Traffic_MultiCore/Environment/Sensors/PlantModel/Object_Sensor_3D/ObjectData/Sensor2/Object_Custom_Values ==
  TrafficObject_Type[] : Inport
  TrafficObject_Type_Data[] : Inport  Port=2
  CUSTOM_SENSOR_OUTPUT : ASM_Traffic_lib/Sensors/Custom_Sensor/CUSTOM_SENSOR_OUTPUT  Tag=ASM_SUBCOMPONENT  ASMProperties=struct('Name','CUSTOM_SENSOR_OUTPUT','Version','5.0','Library','ASM_Traffic_lib')  ASMInstanceName=custom_sensor_output  ASMInstanceID=5
      settings: AttributesFormatString=Instance Name: %<ASMInstanceName>\nInstance ID: %<ASMInstanceID>
  CUSTOM_SENSOR_OUTPUT1 : ASM_Traffic_lib/Sensors/Custom_Sensor/CUSTOM_SENSOR_OUTPUT  Tag=ASM_SUBCOMPONENT  ASMProperties=struct('Name','CUSTOM_SENSOR_OUTPUT','Version','5.0','Library','ASM_Traffic_lib')  ASMInstanceName=custom_sensor_output  ASMInstanceID=6
      settings: AttributesFormatString=Instance Name: %<ASMInstanceName>\nInstance ID: %<ASMInstanceID>
  CUSTOM_SENSOR_OUTPUT2 : ASM_Traffic_lib/Sensors/Custom_Sensor/CUSTOM_SENSOR_OUTPUT  Tag=ASM_SUBCOMPONENT  ASMProperties=struct('Name','CUSTOM_SENSOR_OUTPUT','Version','5.0','Library','ASM_Traffic_lib')  ASMInstanceName=custom_sensor_output  ASMInstanceID=7
      settings: AttributesFormatString=Instance Name: %<ASMInstanceName>\nInstance ID: %<ASMInstanceID>
  Terminator : Terminator
  Terminator1 : Terminator
  Terminator2 : Terminator
  Vectorize_Signals : Subsystem
  "[11:15]" : Selector  IndexOptions=Index vector (dialog)  Indices=[11:15]  OutputSizes=1
  "[1:5]" : Selector  IndexOptions=Index vector (dialog)  Indices=[1:5]  OutputSizes=1
  "[6:10]" : Selector  IndexOptions=Index vector (dialog)  Indices=[6:10]  OutputSizes=1
  ASMSignalBus : Outport  VectorParamsAs1DForOutWhenUnconnected=off
  Object_Custom_Values[] : Outport  Port=2  VectorParamsAs1DForOutWhenUnconnected=off
  wires:
  "[11:15]"/1 -> CUSTOM_SENSOR_OUTPUT2/1
  "[1:5]"/1 -> CUSTOM_SENSOR_OUTPUT/1
  TrafficObject_Type_Data[]/1 -> CUSTOM_SENSOR_OUTPUT1/2, CUSTOM_SENSOR_OUTPUT2/2, CUSTOM_SENSOR_OUTPUT/2
  TrafficObject_Type[]/1 -> "[11:15]"/1, "[6:10]"/1, "[1:5]"/1
  "[6:10]"/1 -> CUSTOM_SENSOR_OUTPUT1/1
  CUSTOM_SENSOR_OUTPUT/1 -> Terminator/1
  CUSTOM_SENSOR_OUTPUT1/1 -> Terminator1/1
  CUSTOM_SENSOR_OUTPUT2/1 -> Terminator2/1
  CUSTOM_SENSOR_OUTPUT/2 -> Vectorize_Signals/1(SensorOutput1)
  Vectorize_Signals/1(Vectorized_Custom_Values) -> Object_Custom_Values[]/1, ASMSignalBus/1
  CUSTOM_SENSOR_OUTPUT1/2 -> Vectorize_Signals/2(SensorOutput2)
  CUSTOM_SENSOR_OUTPUT2/2 -> Vectorize_Signals/3(SensorOutput3)

== system ASM_Traffic_MultiCore/Environment/Sensors/PlantModel/Object_Sensor_3D/ObjectData/Sensor3/ASMSignalCollector ==
  Object_Positions : Inport
  Object_Properties_Box : Inport  Port=2
  Object_Custom_Values : Inport  Port=3
  Bus Creator1 : BusCreator  Inputs=3
  Bus Selector : BusSelector  OutputSignals=Object_Positions
  Bus Selector1 : BusSelector  OutputSignals=Object_Properties_Box
  ASMSignalBus : Outport  VectorParamsAs1DForOutWhenUnconnected=off
  wires:
  Object_Positions/1 -> Bus Selector/1
  Object_Custom_Values/1 -> Bus Creator1/3
  Bus Creator1/1 -> ASMSignalBus/1  "ObjectData"
  Object_Properties_Box/1 -> Bus Selector1/1
  Bus Selector/1 -> Bus Creator1/1  "<Object_Positions>"
  Bus Selector1/1 -> Bus Creator1/2  "<Object_Properties_Box>"

== system ASM_Traffic_MultiCore/Environment/Sensors/PlantModel/Object_Sensor_3D/ObjectData/Sensor3/GetFellowPositionVector ==
  <FellowPositions> : Inport
  Bus Selector11 : BusSelector  OutputSignals=Pos_Fellows_MainPnt_CoorSys_E[x;y;z][m].Pos_x_Fellows[m],Pos_Fellows_MainPnt_CoorSys_E[x;y;z][m].Pos_y_Fellows[m],Pos_Fellows_MainPnt_CoorSys_E[x;y;z][m].Pos_z_Fellows[m],Angle_Fellows[x;y;z][deg].Angle_Roll_Fellows[deg],Angle_Fellows[x;y;z][deg].Angle_Pitch_Fellows[deg],Angle_Fellows[x;y;z][deg].Angle_Yaw_Fellows[deg]
  Mux1 : Mux  Inputs=3
  Mux2 : Mux  Inputs=3
  Pos_Fellows_MainPnt_CoorSys_E[x;y;z][m] : Outport  VectorParamsAs1DForOutWhenUnconnected=off
  Angle_Fellows[deg] : Outport  Port=2  VectorParamsAs1DForOutWhenUnconnected=off
  wires:
  Mux2/1 -> Pos_Fellows_MainPnt_CoorSys_E[x;y;z][m]/1  "Pos_Fellows_MainPnt_CoorSys_E[x;y;z][m]"
  Mux1/1 -> Angle_Fellows[deg]/1  "Pos_Fellows_MainPnt_CoorSys_E_vec"
  Bus Selector11/4 -> Mux1/1  "<Angle_Roll_Fellows[deg]>"
  Bus Selector11/1 -> Mux2/1  "<Pos_x_Fellows[m]>"
  Bus Selector11/2 -> Mux2/2  "<Pos_y_Fellows[m]>"
  Bus Selector11/6 -> Mux1/3  "<Angle_Yaw_Fellows[deg]>"
  Bus Selector11/5 -> Mux1/2  "<Angle_Pitch_Fellows[deg]>"
  <FellowPositions>/1 -> Bus Selector11/1
  Bus Selector11/3 -> Mux2/3  "<Pos_z_Fellows[m]>"

== system ASM_Traffic_MultiCore/Environment/Sensors/PlantModel/Object_Sensor_3D/ObjectData/Sensor3/Object_Custom_Values ==
  TrafficObject_Type[] : Inport
  TrafficObject_Type_Data[] : Inport  Port=2
  CUSTOM_SENSOR_OUTPUT : ASM_Traffic_lib/Sensors/Custom_Sensor/CUSTOM_SENSOR_OUTPUT  Tag=ASM_SUBCOMPONENT  ASMProperties=struct('Name','CUSTOM_SENSOR_OUTPUT','Version','5.0','Library','ASM_Traffic_lib')  ASMInstanceName=custom_sensor_output  ASMInstanceID=8
      settings: AttributesFormatString=Instance Name: %<ASMInstanceName>\nInstance ID: %<ASMInstanceID>
  CUSTOM_SENSOR_OUTPUT1 : ASM_Traffic_lib/Sensors/Custom_Sensor/CUSTOM_SENSOR_OUTPUT  Tag=ASM_SUBCOMPONENT  ASMProperties=struct('Name','CUSTOM_SENSOR_OUTPUT','Version','5.0','Library','ASM_Traffic_lib')  ASMInstanceName=custom_sensor_output  ASMInstanceID=9
      settings: AttributesFormatString=Instance Name: %<ASMInstanceName>\nInstance ID: %<ASMInstanceID>
  CUSTOM_SENSOR_OUTPUT2 : ASM_Traffic_lib/Sensors/Custom_Sensor/CUSTOM_SENSOR_OUTPUT  Tag=ASM_SUBCOMPONENT  ASMProperties=struct('Name','CUSTOM_SENSOR_OUTPUT','Version','5.0','Library','ASM_Traffic_lib')  ASMInstanceName=custom_sensor_output  ASMInstanceID=10
      settings: AttributesFormatString=Instance Name: %<ASMInstanceName>\nInstance ID: %<ASMInstanceID>
  Terminator : Terminator
  Terminator1 : Terminator
  Terminator2 : Terminator
  Vectorize_Signals : Subsystem
  "[11:15]" : Selector  IndexOptions=Index vector (dialog)  Indices=[11:15]  OutputSizes=1
  "[1:5]" : Selector  IndexOptions=Index vector (dialog)  Indices=[1:5]  OutputSizes=1
  "[6:10]" : Selector  IndexOptions=Index vector (dialog)  Indices=[6:10]  OutputSizes=1
  ASMSignalBus : Outport  VectorParamsAs1DForOutWhenUnconnected=off
  Object_Custom_Values[] : Outport  Port=2  VectorParamsAs1DForOutWhenUnconnected=off
  wires:
  CUSTOM_SENSOR_OUTPUT2/2 -> Vectorize_Signals/3(SensorOutput3)
  CUSTOM_SENSOR_OUTPUT1/2 -> Vectorize_Signals/2(SensorOutput2)
  Vectorize_Signals/1(Vectorized_Custom_Values) -> Object_Custom_Values[]/1, ASMSignalBus/1
  CUSTOM_SENSOR_OUTPUT/2 -> Vectorize_Signals/1(SensorOutput1)
  CUSTOM_SENSOR_OUTPUT2/1 -> Terminator2/1
  CUSTOM_SENSOR_OUTPUT1/1 -> Terminator1/1
  CUSTOM_SENSOR_OUTPUT/1 -> Terminator/1
  "[6:10]"/1 -> CUSTOM_SENSOR_OUTPUT1/1
  TrafficObject_Type[]/1 -> "[1:5]"/1, "[6:10]"/1, "[11:15]"/1
  TrafficObject_Type_Data[]/1 -> CUSTOM_SENSOR_OUTPUT2/2, CUSTOM_SENSOR_OUTPUT1/2, CUSTOM_SENSOR_OUTPUT/2
  "[1:5]"/1 -> CUSTOM_SENSOR_OUTPUT/1
  "[11:15]"/1 -> CUSTOM_SENSOR_OUTPUT2/1
